simulink model "Efeitos_da_Amostragem_2_2024a"  (R2024a)
settings: Solver=VariableStepAuto  StartTime=0.0  StopTime=inf  MaxStep=1e-5  RelTol=1e-3
libraries: dspsnks4 x2, dspfdesign x1
settings Model: Creator=rcard  LastModifiedBy=cardo
settings OptimizationCC: ReuseModelBlockBuffer=off
settings RTWCC: GPUComputeCapability=3.5
settings ConfigComp: CovBoundaryAbsTol=1.0e-5

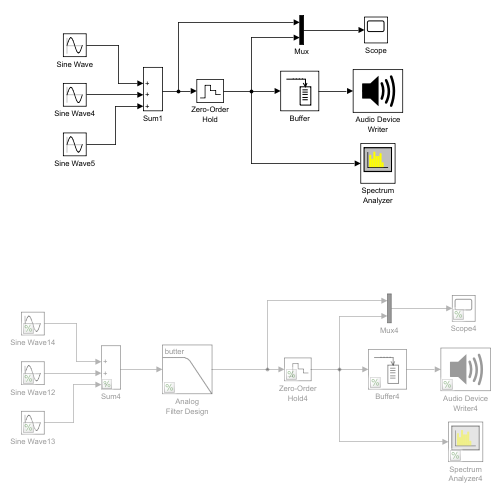
[thumbnail: Simulink's stored preview of the top-level diagram]
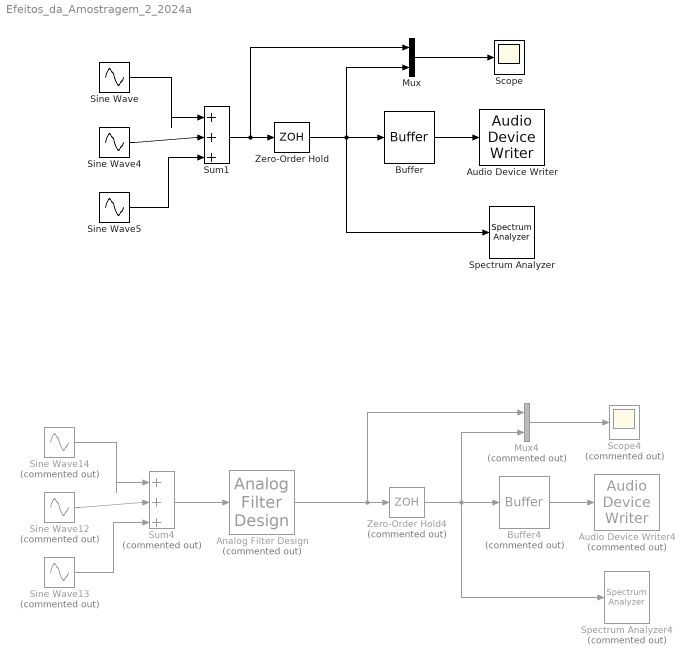
== system Efeitos_da_Amostragem_2_2024a ==
  Analog Filter Design : dspfdesign/Analog Filter Design  Commented=on  method=Butterworth  filttype=Lowpass  N=4  Wlo=2*pi*600  Whi=80  Rp=2  Rs=40
  Audio Device Writer : dspsnks4/Audio Device Writer  Driver=DirectSound  Device=Default  InheritSampleRate=on  SampleRate=44100  BitDepth=24-bit integer  BufferSize=4096  NumBuffers=10  DefaultOutputChannelMapping=on  OutputChannelMapping=1:2  OutputNumUnderrunSamples=off  DriverIdx=1  DeviceWarnFlag=''
  Audio Device Writer4 : dspsnks4/Audio Device Writer  Commented=on  Driver=DirectSound  Device=Default  InheritSampleRate=on  SampleRate=44100  BitDepth=24-bit integer  BufferSize=4096  NumBuffers=10  DefaultOutputChannelMapping=on  OutputChannelMapping=1:2  OutputNumUnderrunSamples=off  DriverIdx=1  DeviceWarnFlag=''
  Buffer : Buffer  N=128  OutputFrames=off
  Buffer4 : Buffer  Commented=on  N=128  OutputFrames=off
  Mux : Mux  Inputs=2
  Mux4 : Mux  Commented=on  Inputs=2
  Scope : Scope
  Scope4 : Scope  Commented=on
  Sine Wave : Sin  Frequency=2*pi*500  Phase=pi/2  SampleTime=0
  Sine Wave12 : Sin  Commented=on  Frequency=2*pi*6000  Phase=pi/2  SampleTime=0
  Sine Wave13 : Sin  Commented=on  Frequency=2*pi*7000  Phase=pi/2  SampleTime=0
  Sine Wave14 : Sin  Commented=on  Frequency=2*pi*500  Phase=pi/2  SampleTime=0
  Sine Wave4 : Sin  Frequency=2*pi*6000  Phase=pi/2  SampleTime=0
  Sine Wave5 : Sin  Frequency=2*pi*7000  Phase=pi/2  SampleTime=0
  Spectrum Analyzer : SpectrumAnalyzer  WindowPosition=[1282.000000,50.000000,1277.000000,1361.000000,]  ScopeFrameLocation=window  ViewType=Spectrum and spectrogram  SampleRate=2500  PlotAsTwoSidedSpectrum=off  AxesScaling=Manual  Span=24000  CenterFrequency=12000  StartFrequency=0  StopFrequency=1250  AveragingMethod=Exponential  ReferenceLoad=50  YLimits=[-59.4018 27.6706]  ColorLimits=[-59.4018 27.6706]  SelectedToolstripTab=spectrumAnalyzerToolstrip.spectrumTab  AllowFFTLengthLessThanSamplesPerUpdate=on
  Spectrum Analyzer4 : SpectrumAnalyzer  Commented=on  WindowPosition=[1463.000000,48.000000,1048.000000,936.000000,]  Visible=on  ScopeFrameLocation=window  ViewType=Spectrum and spectrogram  SampleRate=2500  PlotAsTwoSidedSpectrum=off  AxesScaling=Manual  Span=24000  CenterFrequency=12000  StartFrequency=0  StopFrequency=1250  AveragingMethod=Exponential  ReferenceLoad=50  YLimits=[-88.6002 20.9195]  ColorLimits=[-88.6002 20.9195]  SelectedToolstripTab=spectrumAnalyzerToolstrip.spectrumTab  AllowFFTLengthLessThanSamplesPerUpdate=on
  Sum1 : Sum  Inputs=|+++
  Sum4 : Sum  Commented=on  Inputs=|+++
  Zero-Order Hold : ZeroOrderHold  SampleTime=1/5000
  Zero-Order Hold4 : ZeroOrderHold  Commented=on  SampleTime=1/5000
  wires:
  Zero-Order Hold/1 -> Spectrum Analyzer/1, Mux/2, Buffer/1
  Buffer/1 -> Audio Device Writer/1
  Mux/1 -> Scope/1
  Sum1/1 -> Mux/1, Zero-Order Hold/1
  Sine Wave/1 -> Sum1/1
  Sine Wave4/1 -> Sum1/2
  Sine Wave5/1 -> Sum1/3
  Mux4/1 -> Scope4/1
  Sine Wave12/1 -> Sum4/2
  Zero-Order Hold4/1 -> Spectrum Analyzer4/1, Mux4/2, Buffer4/1
  Sine Wave14/1 -> Sum4/1
  Sine Wave13/1 -> Sum4/3
  Sum4/1 -> Analog Filter Design/1
  Buffer4/1 -> Audio Device Writer4/1
  Analog Filter Design/1 -> Mux4/1, Zero-Order Hold4/1
